simulink model "First_order_loop"  (R2025a)
settings: Solver=VariableStepAuto  StartTime=0.0  StopTime=10.0  RelTol=1e-3
libraries: simulink x2
settings Model: Creator=庞亚宸  LastModifiedBy=庞亚宸

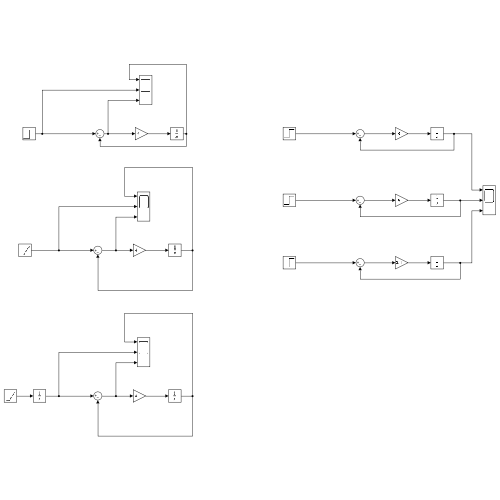
[thumbnail: Simulink's stored preview of the top-level diagram]
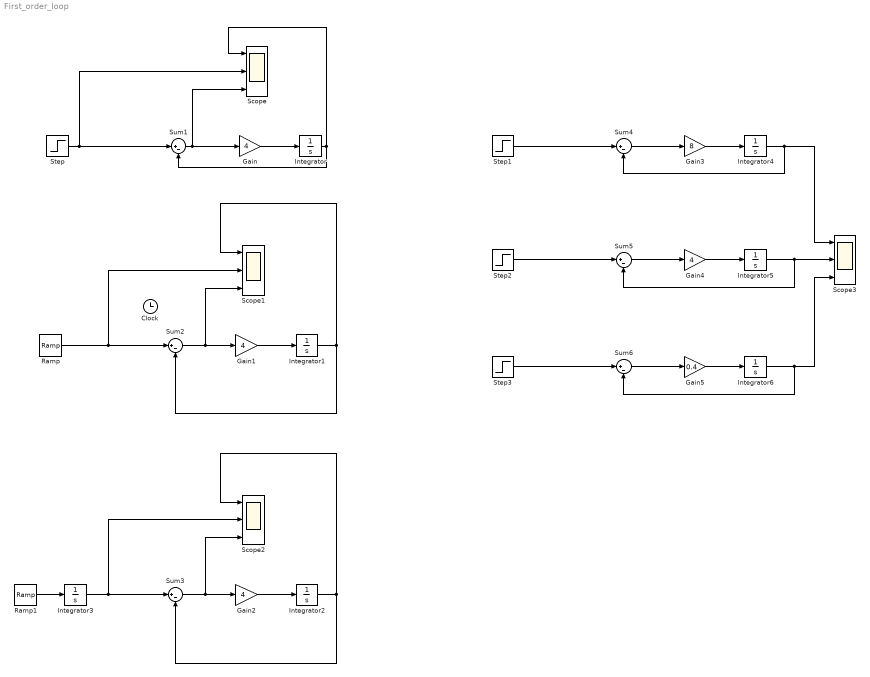
== system First_order_loop ==
  Gain{,1..2,4} (4 alike) : Gain  Gain=4
  Gain3 : Gain  Gain=8
  Gain5 : Gain  Gain=0.4
  Integrator{,1..6} (7 alike) : Integrator
  Ramp : simulink/Sources/Ramp  slope=1  start=0  InitialOutput=0
  Ramp1 : simulink/Sources/Ramp  slope=1  start=0  InitialOutput=0
  Scope{,1..3} (4 alike) : Scope  NumInputPorts=3
      Scope settings: ActiveDisplayYMinimum=-0.12499999999999996  ActiveDisplayYMaximum=1.1249999999999998
      Scope1 settings: ActiveDisplayYMinimum=-1.2187499999999998  ActiveDisplayYMaximum=10.96875
      Scope2 settings: ActiveDisplayYMinimum=-5.9453125000000044  ActiveDisplayYMaximum=53.50781250000005  DataLoggingVariableName=ScopeData2
      Scope3 settings: ActiveDisplayYMinimum=-0.12499999999999997  ActiveDisplayYMaximum=1.125  DataLoggingVariableName=ScopeData3
  Step{,1..3} (4 alike) : Step  Time=0  SampleTime=0
  Sum{1..6} (6 alike) : Sum  Inputs=|+-
  Clock : Clock
      settings: IOType=siggen
  wires:
  Sum1/1 -> Scope/3, Gain/1
  Gain/1 -> Integrator/1
  Step/1 -> Scope/2, Sum1/1
  Integrator/1 -> Scope/1, Sum1/2
  Integrator1/1 -> Scope1/1, Sum2/2
  Ramp/1 -> Scope1/2, Sum2/1
  Sum2/1 -> Scope1/3, Gain1/1
  Gain1/1 -> Integrator1/1
  Ramp1/1 -> Integrator3/1
  Gain2/1 -> Integrator2/1
  Integrator2/1 -> Scope2/1, Sum3/2
  Sum3/1 -> Scope2/3, Gain2/1
  Integrator3/1 -> Scope2/2, Sum3/1
  Integrator4/1 -> Sum4/2, Scope3/1
  Step1/1 -> Sum4/1
  Sum4/1 -> Gain3/1
  Gain3/1 -> Integrator4/1
  Sum5/1 -> Gain4/1
  Step2/1 -> Sum5/1
  Gain4/1 -> Integrator5/1
  Integrator5/1 -> Sum5/2, Scope3/2
  Integrator6/1 -> Scope3/3, Sum6/2
  Gain5/1 -> Integrator6/1
  Step3/1 -> Sum6/1
  Sum6/1 -> Gain5/1
